simulink model "DroopControl"  (R2025b)
settings: Solver=VariableStepAuto  StartTime=0.0  StopTime=0.3  MaxStep=1/20e3/100  RelTol=1e-3
InitFcn:
  | fs = 20000;
  | Ts = 1/fs;
  | I2B = 10;
  | UB = 20;
  | freq0 = 50;
  | freqc = 0.29999999999999999;
  | w0 = 2*pi*freq0;
  | wc = 2*pi*freqc;
  | I2_Kp = 3.023;
  | I2_Kr = 16.36;
  | Uc_Kp = 0.010579843316015665;
  | Uc_Kr = 0.56544574743993026;
  | I1_Kpi = 1.73;
  | UDC = 48;
  | Ic_Kd = 0;
  | Ts2 = 1/500;
  | 
  | %% 20V / 12A droop-grid configuration
  | % wc_grid is separate from the existing QPR parameter wc.
  | Grid_Condition = 'STRONG'; % STRONG / WEAK_INDUCTIVE / WEAK_RESISTIVE
  | fn = 50;
  | wn = 2*pi*fn;
  | E0 = 20; % phase-voltage peak, V
  | I_base = 12; % current peak, A
  | S_inv = 1.5*E0*I_base;
  | Z_base = E0/I_base;
  | switch Grid_Condition
  |     case 'STRONG'
  |         SCR = 10;
  |         XR_ratio = 5;
  |         Sn = 10*S_inv;
  |         delta_f_max = 0.2;
  |         delta_E_max = 0.02*E0;
  |         grid_wc = 25; % power-filter cutoff, rad/s
  |     case 'WEAK_INDUCTIVE'
  |         SCR = 1.5;
  |         XR_ratio = 3;
  |         Sn = 1.5*S_inv;
  |         delta_f_max = 1.5;
  |         delta_E_max = 0.10*E0;
  |         grid_wc = 120;
  |     case 'WEAK_RESISTIVE'
  |         SCR = 1.5;
  |         XR_ratio = 1;
  |         Sn = 1.5*S_inv;
  |         delta_f_max = 1.5;
  |         delta_E_max = 0.10*E0;
  |         grid_wc = 120;
  |     otherwise
  |         error('DroopGrid:InvalidCondition','Unknown Grid_Condition: %s',Grid_Condition);
  | end
  | Z_grid = Z_base/SCR;
  | Rg_val = Z_grid/sqrt(1+XR_ratio^2);
  | Lg_val = Rg_val*XR_ratio/wn;
  | grid_mp = 2*pi*delta_f_max/Sn;
  | grid_nq = delta_E_max/Sn;
  | grid_p0 = 0;
  | grid_q0 = 0;
  | Ts_ctrl = 1e-4; % actual droop-grid update period, 10 kHz
  | 
  | ... (+21 lines)
model workspace (MAT data in the model file):
  CurrentTestFinalPeak = 0.3
  CurrentTestInitialPeak = 0.1
  CurrentTestSignedStepTime = 0.03
libraries: nesl_utility x31, fl_lib x28, ee_lib x27, simulink x1, eePowerMeasurement x1
(part 2 of 2)

== system DroopControl/I2处理+标幺化/Clark ==
  abc : Inport
  B : Inport  Port=2
  MATLAB Function1 : MATLAB Function  TreatAsAtomicUnit=on
  α : Outport
  β : Outport  Port=2
  wires:
  MATLAB Function1/1(alpha) -> α/1
  abc/1 -> MATLAB Function1/1(abc)
  MATLAB Function1/2(beta) -> β/1
  B/1 -> MATLAB Function1/2(B)

== system DroopControl/数字滤波器+标幺化/Clark1 ==
  abc : Inport
  B : Inport  Port=2
  MATLAB Function1 : MATLAB Function  TreatAsAtomicUnit=on
  α : Outport
  β : Outport  Port=2
  Out3 : Outport  Port=3
  wires:
  MATLAB Function1/1(alpha) -> α/1
  abc/1 -> MATLAB Function1/1(abc)
  MATLAB Function1/2(beta) -> β/1
  B/1 -> MATLAB Function1/2(B)

== system DroopControl/电容线电压处理+标幺化/Clark ==
  abc : Inport
  B : Inport  Port=2
  MATLAB Function1 : MATLAB Function  TreatAsAtomicUnit=on
  α : Outport
  β : Outport  Port=2
  Out3 : Outport  Port=3
  wires:
  B/1 -> MATLAB Function1/2(B)
  MATLAB Function1/2(beta) -> β/1
  abc/1 -> MATLAB Function1/1(abc)
  MATLAB Function1/1(alpha) -> α/1

== system DroopControl/网侧线电压处理+标幺化/Clark ==
  abc : Inport
  B : Inport  Port=2
  MATLAB Function1 : MATLAB Function  TreatAsAtomicUnit=on
  α : Outport
  β : Outport  Port=2
  Out3 : Outport  Port=3
  wires:
  MATLAB Function1/1(alpha) -> α/1
  abc/1 -> MATLAB Function1/1(abc)
  MATLAB Function1/2(beta) -> β/1
  B/1 -> MATLAB Function1/2(B)

== matlab function DroopControl/I2处理+标幺化/Clark/MATLAB Function1 ==
  settings: updateMethod=DISCRETE
  data: abc input; alpha output; beta output; B input
function [alpha, beta] = abc2alphabeta_mux(abc, B)
%#codegen
% ABC2ALPHABETA_MUX  输入 mux 后的 3 通道信号，输出 alpha-beta
%   abc : [3 x N] 矩阵，第 1/2/3 行分别为 a/b/c
%   alpha, beta : [1 x N] 行向量（可直接接 Scope / Mux 输出）
%
%   Simulink 用法：
%     Mux (3 inputs) --> MATLAB Function --> 输出 alpha, beta

    % 按行取出三相，兼容 [3x1] 和 [3xN]
    a = abc(1, :);
    b = abc(2, :);
    c = abc(3, :);

    K = 2/3;   % 等幅值 Clarke 系数；改 sqrt(2/3) 为等功率

    alpha = K * ( a - 0.5*b - 0.5*c ) / B;
    beta  = K * ( (sqrt(3)/2) * (b - c) ) / B;
end

== matlab function DroopControl/Triggered Subsystem1/MATLAB Function1 ==
  settings: updateMethod=DISCRETE
  data: e input; u_r_prev1 input; u_r_prev2 input; e_prev1 input; e_prev2 input; Kp input; Kr input; wc input; w0 input; u_out output; u_r_state output; Ts input
function [u_out, u_r_state] = QPR_Controller(e, u_r_prev1, u_r_prev2, e_prev1, e_prev2, Kp, Kr, wc, w0, Ts)
% QPR电压外环控制器（离散化实现，Tustin变换）
% 输入：
%   e         : 当前时刻电压误差 (v_ref - v_cap)
%   u_r_prev1 : 谐振项上一时刻输出 u_r(k-1)
%   u_r_prev2 : 谐振项上上时刻输出 u_r(k-2)
%   e_prev1   : 上一时刻误差 e(k-1)
%   e_prev2   : 上上时刻误差 e(k-2)
%   Kp, Kr    : 比例系数、谐振系数
%   wc        : 截止频率 (rad/s)
%   w0        : 谐振频率 (rad/s)，如 2*pi*50
%   Ts        : 采样周期 (s)
%
% 输出：
%   u_out     : QPR控制器输出
%   u_r_state : 谐振项当前输出（用于下一时刻状态更新）

% 计算离散化系数
xi = 2 * wc;
den = 4 + 2*xi*Ts + w0^2*Ts^2;

a1 = 2 * (w0^2*Ts^2 - 4) / den;
a2 = (4 - 2*xi*Ts + w0^2*Ts^2) / den;
b0 = 4 * Kr * xi * Ts / den;
b1 = 0;
b2 = -b0;

% 谐振项差分方程迭代
u_r = b0*e + b1*e_prev1 + b2*e_prev2 - a1*u_r_prev1 - a2*u_r_prev2;

% 比例项 + 谐振项
u_out = Kp * e + u_r;

% 输出当前谐振项状态（供下一周期使用）
u_r_state = u_r;
end

== matlab function DroopControl/I1处理+标幺化/Clark/MATLAB Function1 ==
  settings: updateMethod=DISCRETE
  data: abc input; alpha output; beta output; B input
function [alpha, beta] = abc2alphabeta_mux(abc, B)
%#codegen
% ABC2ALPHABETA_MUX  输入 mux 后的 3 通道信号，输出 alpha-beta
%   abc : [3 x N] 矩阵，第 1/2/3 行分别为 a/b/c
%   alpha, beta : [1 x N] 行向量（可直接接 Scope / Mux 输出）
%
%   Simulink 用法：
%     Mux (3 inputs) --> MATLAB Function --> 输出 alpha, beta

    % 按行取出三相，兼容 [3x1] 和 [3xN]
    a = abc(1, :);
    b = abc(2, :);
    c = abc(3, :);

    K = 2/3;   % 等幅值 Clarke 系数；改 sqrt(2/3) 为等功率

    alpha = K * ( a - 0.5*b - 0.5*c ) / B;
    beta  = K * ( (sqrt(3)/2) * (b - c) ) / B;
end

== matlab function DroopControl/I1处理+标幺化/MATLAB Function1 ==
  settings: updateMethod=DISCRETE
  data: y output; real input
function y = fcn(real)
   y = real;
end

== matlab function DroopControl/DroopGridEngine/MATLAB Function1 ==
  settings: updateMethod=DISCRETE  sampleTime=Ts_ctrl
  data: Vabc input; Iabc input; E0 input; wn input; mp input; nq input; wc input; P0 input; Q0 input; v_cmd_abc output; Ts input
function v_cmd_abc = Simscape_Droop_Grid(Vabc, Iabc, E0, wn, mp, nq, wc, P0, Q0, Ts)
%#codegen
% 输入:
%   Vabc      : 采样相电压 [va; vb; vc] (V)
%   Iabc      : 采样输出电流 [ia; ib; ic] (A)
%   E0, wn    : 额定相电压幅值 (V) 与工频角频率 (rad/s)
%   mp, nq    : 下垂系数
%   wc        : 功率低通滤波截止角频率 (rad/s)
%   P0, Q0    : 基准工作功率
%   Ts        : 控制步长 (s)
% 输出:
%   v_cmd_abc : 输送给受控源的参考相电压 [va*; vb*; vc*]

persistent P_filt Q_filt theta
if isempty(P_filt)
    P_filt = 0;
    Q_filt = 0;
    theta = 0;
end

%% 1. 瞬时功率计算 (等幅值 Clarke 变换)
va = Vabc(1); vb = Vabc(2); vc = Vabc(3);
ia = Iabc(1); ib = Iabc(2); ic = Iabc(3);

% Clarke 变换 (2/3 系数)
v_alpha = (2/3) * (va - 0.5 * vb - 0.5 * vc);
v_beta  = (2/3) * (sqrt(3)/2 * vb - sqrt(3)/2 * vc);

i_alpha = (2/3) * (ia - 0.5 * ib - 0.5 * ic);
i_beta  = (2/3) * (sqrt(3)/2 * ib - sqrt(3)/2 * ic);

% 瞬时有功与无功
p_inst = 1.5 * (v_alpha * i_alpha + v_beta * i_beta);
q_inst = 1.5 * (v_beta  * i_alpha - v_alpha * i_beta);

%% 2. 功率滤波 (消除开关纹波并模拟系统惯性)
alpha = (wc * Ts) / (1 + wc * Ts);
P_filt = (1 - alpha) * P_filt + alpha * p_inst;
Q_filt = (1 - alpha) * Q_filt + alpha * q_inst;

%% 3. 下垂特性
w_grid = wn - mp * (P_filt - P0);
E_grid = E0 - nq * (Q_filt - Q0);

% 幅值软限幅防击穿
if E_grid < 0.7 * E0
    E_grid = 0.7 * E0;
elseif E_grid > 1.3 * E0
    E_grid = 1.3 * E0;
end

%% 4. 相角积分
theta = theta + w_grid * Ts;
if theta >= 2 * pi
    theta = theta - 2 * pi;
elseif theta < 0
    theta = theta + 2 * pi;
end

%% 5. 合成三相调制波
v_cmd_abc = [
    E_grid * cos(theta);
    E_grid * cos(theta - 2*pi/3);
    E_grid * cos(theta + 2*pi/3)
];
end

== matlab function DroopControl/Droop Controll /MATLAB Function1 ==
  settings: updateMethod=DISCRETE
  data: v_cap_alpha input; v_cap_beta input; i_inv_alpha input; i_inv_beta input; v_grid_alpha input; v_grid_beta input; w0 input; E0 input; mp input; nq input; wc input; v_alpha_ref output; v_beta_ref output; Ts input; P_filt output; Q_filt output; w_out output; breaker_cmd output
function [v_alpha_ref, v_beta_ref, P_filt, Q_filt, w_out, breaker_cmd] = Droop_Control_Sync( ...
    v_cap_alpha,  v_cap_beta,  ... % 【输入1】逆变器输出电容侧电压 (αβ 坐标系)
    i_inv_alpha,  i_inv_beta,  ... % 【输入2】逆变器输出侧网侧/负载电流 (αβ 坐标系)
    v_grid_alpha, v_grid_beta, ... % 【输入3】外部主电网侧母线电压 (αβ 坐标系)
    w0, E0, mp, nq, wc, Ts)
%#codegen
% =========================================================================
% 输入说明:
%   v_cap_alpha, v_cap_beta   : [输出电容侧] 逆变器 LC 滤波电容两端电压 (V)
%   i_inv_alpha, i_inv_beta   : [输出电容侧] 流向断路器/负载的输出电流 (A)
%   v_grid_alpha, v_grid_beta : [外部电网侧] 三相断路器外侧电网母线电压 (V)
%   w0, E0                    : 额定角频率 (rad/s) 与额定相电压幅值 (V)
%   mp, nq                    : 有功/无功下垂系数
%   wc                        : 功率低通滤波截止角频率 (rad/s)
%   Ts                        : 控制步长 (s)
% 输出说明:
%   v_alpha_ref, v_beta_ref   : QPR 电压内环参考电压 (αβ 轴)
%   P_filt, Q_filt            : 滤波后的有功/无功功率
%   f_out                     : 逆变器当前输出频率 (Hz)
%   breaker_cmd               : 三相断路器合闸指令 (3x1 向量: [cmd_a; cmd_b; cmd_c])
%                               0 = 断开 (未同步/离网), 1 = 合闸导通 (同步完成)
% =========================================================================

%% 内部状态保持
persistent P_prev Q_prev theta_prev
persistent sync_integ sync_ok_counter is_breaker_closed

if isempty(P_prev)
    P_prev = 0;
    Q_prev = 0;
    theta_prev = 0;
    sync_integ = 0;
    sync_ok_counter = 0;
    is_breaker_closed = false;
end

%% 1. 瞬时功率计算 (基于输出电容侧电压与输出电流)
p_inst = 1.5 * (v_cap_alpha * i_inv_alpha + v_cap_beta * i_inv_beta);
q_inst = 1.5 * (v_cap_beta * i_inv_alpha - v_cap_alpha * i_inv_beta);

%% 2. 功率一阶低通滤波
alpha = (wc * Ts) / (1 + wc * Ts);
P_filt = (1 - alpha) * P_prev + alpha * p_inst;
Q_filt = (1 - alpha) * Q_prev + alpha * q_inst;
P_prev = P_filt;
Q_prev = Q_filt;

% 3. Independent inverter: presynchronization and closure disabled.
w_sync = 0;
E_sync = 0;

%% 4. 下垂方程叠加与参考频率/幅值生成
% 频率计算 (并网前叠加上 w_sync 进行调相；并网后 w_sync 归零，由 -mp*P 维持功角自同步)
w_out = (w0 - mp * P_filt) + w_sync;

% 幅值计算 (并网前叠加上 E_sync 消除压差；并网后回归标准下垂)
E_out = (E0 - nq * Q_filt) + E_sync;

% 基础安全限幅
if E_out < 0.8 * E0
    E_out = 0.8 * E0;
elseif E_out > 1.2 * E0
    E_out = 1.2 * E0;
end

%% 5. 相角自累加积分
theta = theta_prev + w_out * Ts;
if theta >= 2 * pi
    theta = theta - 2 * pi;
elseif theta < 0
    theta = theta + 2 * pi;
end
theta_prev = theta;

%% 6. 合成 αβ 轴参考电压 (送入 QPR 电压内环)
v_alpha_ref = E_out * cos(theta);
v_beta_ref  = E_out * sin(theta);

%% 7. 组装三相断路器动作信号
if is_breaker_closed
    % 准同期条件满足，输出合闸指令 (给 1 触发导通/合闸)
    breaker_cmd = [0; 0; 0];
else
    % 预同步中或离网状态，保持断开
    breaker_cmd = [1; 1; 1];
end

end

== matlab function DroopControl/电容线电压处理+标幺化/Clark/MATLAB Function1 ==
  settings: updateMethod=DISCRETE
  data: abc input; alpha output; beta output; B input
function [alpha, beta] = abc2alphabeta_mux(abc, B)
%#codegen
% ABC2ALPHABETA_MUX  输入 mux 后的 3 通道信号，输出 alpha-beta
%   abc : [3 x N] 矩阵，第 1/2/3 行分别为 a/b/c
%   alpha, beta : [1 x N] 行向量（可直接接 Scope / Mux 输出）
%
%   Simulink 用法：
%     Mux (3 inputs) --> MATLAB Function --> 输出 alpha, beta

    % 按行取出三相，兼容 [3x1] 和 [3xN]
    a = abc(1, :);
    b = abc(2, :);
    c = abc(3, :);

    K = 2/3;   % 等幅值 Clarke 系数；改 sqrt(2/3) 为等功率

    alpha = K * ( a - 0.5*b - 0.5*c ) / B;
    beta  = K * ( (sqrt(3)/2) * (b - c) ) / B;
end

== matlab function DroopControl/电容线电压处理+标幺化/MATLAB Function1 ==
  settings: updateMethod=DISCRETE
  data: Uabc output; U_line input
function Uabc = line2phase(U_line)
%#codegen
% 输入 U_line: [Uab; Ubc; Uac]  3x1
% 输出 Uabc : [Ua;  Ub;  Uc ]  3x1

Uab = U_line(1);
Ubc = U_line(2);
Uac = U_line(3);

Ua = ( Uab + Uac) / 3;
Ub = ( Ubc - Uab) / 3;
Uc = -(Ubc + Uac) / 3;

Uabc = [Ua; Ub; Uc];
end

== matlab function DroopControl/Triggered Subsystem2/MATLAB Function1 ==
  settings: updateMethod=DISCRETE
  data: i1_alpha_ref input; i1_beta_ref input; i1_alpha input; i1_beta input; uc_alpha input; uc_beta input; Kpi input; u_alpha_ref output; u_beta_ref output
function [u_alpha_ref, u_beta_ref] = current_loop( ...
    i1_alpha_ref, i1_beta_ref, ...
    i1_alpha, i1_beta, ...
    uc_alpha, uc_beta, Kpi)
%#codegen
% i1 比例电流环，带 uc 电压前馈，不加 ic 阻尼
%
% 电流单位：A
% 电压单位：V
% Kpi 单位：V/A（欧姆）
% 输出：送往调制器的 alpha、beta 电压指令

% 电流误差
e_alpha = i1_alpha_ref - i1_alpha;
e_beta  = i1_beta_ref  - i1_beta;

% 比例控制 + 电容电压前馈
u_alpha_ref = Kpi * e_alpha + uc_alpha;
u_beta_ref  = Kpi * e_beta  + uc_beta;

end

== matlab function DroopControl/α,β转SVPWM调制波1/MATLAB Function1 ==
  settings: updateMethod=DISCRETE
  data: valpha_pu input; A_SVM output; B_SVM output; vbeta_pu input; C_SVM output; Vbase input; Udc input
function [A_SVM, B_SVM, C_SVM] = ...
    svpwm_simple_pu(valpha_pu, vbeta_pu, Vbase, Udc)
%#codegen

% 母线电压尚未建立时，输出零线电压指令
if Udc <= 1e-6
    A_SVM = 0;
    B_SVM = 0;
    C_SVM = 0;
    return;
end

% 将控制器输出恢复为实际电压
Va = valpha_pu * Vbase;
Vb = vbeta_pu  * Vbase;

% 反 Clarke 变换
v = [Va, (-Va + sqrt(3)*Vb)/2, ...
         (-Va - sqrt(3)*Vb)/2];

% 超出母线可实现范围时，等比例缩小电压矢量
span = max(v) - min(v);
if span > Udc
    v = v * (Udc / span);
end

% 零序注入，转换为 0～1 上管占空比
v0 = (max(v) + min(v)) / 2;
d = 0.5 + (v - v0) / Udc;
d = min(max(d, 0), 1);

A_SVM = 2*d(1)-1;
B_SVM = 2*d(2)-1;
C_SVM = 2*d(3)-1;
end
% Average converter ModWave uses signed modulation m=2*d-1.

== matlab function DroopControl/数字滤波器+标幺化/Clark1/MATLAB Function1 ==
  settings: updateMethod=DISCRETE
  data: abc input; alpha output; beta output; B input
function [alpha, beta] = abc2alphabeta_mux(abc, B)
%#codegen
% ABC2ALPHABETA_MUX  输入 mux 后的 3 通道信号，输出 alpha-beta
%   abc : [3 x N] 矩阵，第 1/2/3 行分别为 a/b/c
%   alpha, beta : [1 x N] 行向量（可直接接 Scope / Mux 输出）
%
%   Simulink 用法：
%     Mux (3 inputs) --> MATLAB Function --> 输出 alpha, beta

    % 按行取出三相，兼容 [3x1] 和 [3xN]
    a = abc(1, :);
    b = abc(2, :);
    c = abc(3, :);

    K = 2/3;   % 等幅值 Clarke 系数；改 sqrt(2/3) 为等功率

    alpha = K * ( a - 0.5*b - 0.5*c ) / B;
    beta  = K * ( (sqrt(3)/2) * (b - c) ) / B;
end

== matlab function DroopControl/I2处理+标幺化/MATLAB Function1 ==
  settings: updateMethod=DISCRETE
  data: y output; real input
function y = fcn(real)
   y = real;
end

== matlab function DroopControl/网侧线电压处理+标幺化/MATLAB Function1 ==
  settings: updateMethod=DISCRETE
  data: Uabc output; U_line input
function Uabc = line2phase(U_line)
%#codegen
% 输入 U_line: [Uab; Ubc; Uac]  3x1
% 输出 Uabc : [Ua;  Ub;  Uc ]  3x1

Uab = U_line(1);
Ubc = U_line(2);
Uac = U_line(3);

Ua = ( Uab + Uac) / 3;
Ub = ( Ubc - Uab) / 3;
Uc = -(Ubc + Uac) / 3;

Uabc = [Ua; Ub; Uc];
end

== matlab function DroopControl/数字滤波器+标幺化/MATLAB Function1 ==
  settings: updateMethod=DISCRETE
  data: y output; real input
function y = fcn(real)
   y = real;
end

== matlab function DroopControl/θ转α,β/MATLAB Function1 ==
  settings: updateMethod=DISCRETE
  data: theta input; alpha output; beta output
function [alpha, beta] = theta2alphabeta(theta)
%#codegen
% 输入 theta: 电角度 (rad)
% 输出 alpha, beta: αβ 分量

alpha = cos(theta);
beta  = sin(theta);

end

== matlab function DroopControl/网侧线电压处理+标幺化/Clark/MATLAB Function1 ==
  settings: updateMethod=DISCRETE
  data: abc input; alpha output; beta output; B input
function [alpha, beta] = abc2alphabeta_mux(abc, B)
%#codegen
% ABC2ALPHABETA_MUX  输入 mux 后的 3 通道信号，输出 alpha-beta
%   abc : [3 x N] 矩阵，第 1/2/3 行分别为 a/b/c
%   alpha, beta : [1 x N] 行向量（可直接接 Scope / Mux 输出）
%
%   Simulink 用法：
%     Mux (3 inputs) --> MATLAB Function --> 输出 alpha, beta

    % 按行取出三相，兼容 [3x1] 和 [3xN]
    a = abc(1, :);
    b = abc(2, :);
    c = abc(3, :);

    K = 2/3;   % 等幅值 Clarke 系数；改 sqrt(2/3) 为等功率

    alpha = K * ( a - 0.5*b - 0.5*c ) / B;
    beta  = K * ( (sqrt(3)/2) * (b - c) ) / B;
end

== matlab function DroopControl/SOGI-FLL Subsystem3/MATLAB Function1 ==
  settings: updateMethod=DISCRETE
  data: u input; theta output; omega output; Ts input; locked output
function [theta, omega, locked] = DSOGI_FLL(u, Ts)
% DSOGI-FLL (输入为Mux后的三相电压向量)
% 输入:
%   u  - 3x1 向量 [Ua; Ub; Uc]
%   Ts - 采样周期 (全局变量, 从工作区传入)
% 输出:
%   theta  - 估计相角 (rad)
%   omega  - 估计角频率 (rad/s)
%   locked - 锁相状态 (0=未锁定, 1=已锁定)

% --- 持久变量 (状态) ---
persistent x1_alpha x2_alpha x1_beta x2_beta omega_est lock_cnt
if isempty(x1_alpha)
    x1_alpha = 0; x2_alpha = 0;
    x1_beta  = 0; x2_beta  = 0;
    omega_est = 2*pi*50;   % 初始频率 50 Hz
    lock_cnt  = 0;
end

% --- 参数 ---
k      = sqrt(2);        % SOGI 增益
Gamma  = 100;            % FLL 增益
omega_n = 2*pi*50;       % 额定角频率

% --- 锁定判据参数 ---
eps_lock   = 5;          % 归一化频率误差阈值
lock_hold  = round(0.02 / Ts);   % 连续满足时间 = 20ms 判定为锁定

% --- 1) Clarke 变换 (等幅值) ---
Ua = u(1);  Ub = u(2);  Uc = u(3);
ualpha = (2/3) * (Ua - 0.5*Ub - 0.5*Uc);
ubeta  = (2/3) * ( (sqrt(3)/2)*Ub - (sqrt(3)/2)*Uc );

% --- 2) 限幅保护 ---
omega_est = max(min(omega_est, 2*pi*65), 2*pi*45);

% --- 3) SOGI 离散化 (后向欧拉) ---
% alpha 轴
err_a  = ualpha - x1_alpha;
x1_alpha = x1_alpha + Ts * (k * err_a - x2_alpha) * omega_est;
x2_alpha = x2_alpha + Ts * (x1_alpha * omega_est);

% beta 轴
err_b  = ubeta - x1_beta;
x1_beta = x1_beta + Ts * (k * err_b - x2_beta) * omega_est;
x2_beta = x2_beta + Ts * (x1_beta * omega_est);

% --- 4) 正序分量 (Lyon变换简化形式) ---
v_alpha_pos = 0.5 * (x1_alpha - x2_beta);
v_beta_pos  = 0.5 * (x1_beta  + x2_alpha);

% --- 5) FLL 频率估计 ---
epsilon_f = v_alpha_pos * (x1_beta - ubeta) - v_beta_pos * (x1_alpha - ualpha);

% 归一化 (使 Gamma 与电压幅值无关)
norm_factor = v_alpha_pos^2 + v_beta_pos^2;
if norm_factor > 1e-6
    epsilon_f = epsilon_f / norm_factor;
end
omega_est = omega_est - Gamma * epsilon_f * Ts;

% --- 6) 相角输出 ---
theta = atan2(v_beta_pos, v_alpha_pos);
omega = omega_est;

% --- 7) 锁相完成状态判定 ---
if abs(epsilon_f) < eps_lock
    lock_cnt = lock_cnt + 1;
    if lock_cnt >= lock_hold
        lock_cnt = lock_hold;   % 饱和,防止溢出
    end
else
    lock_cnt = 0;               % 一旦失锁立即清零
end
locked = double(lock_cnt >= lock_hold);

end

== matlab function DroopControl/Triggered Subsystem4/MATLAB Function1 ==
  settings: updateMethod=DISCRETE
  data: e input; u_r_prev1 input; u_r_prev2 input; e_prev1 input; e_prev2 input; Kp input; Kr input; wc input; w0 input; u_out output; u_r_state output; Ts input
function [u_out, u_r_state] = QPR_Controller(e, u_r_prev1, u_r_prev2, e_prev1, e_prev2, Kp, Kr, wc, w0, Ts)
% QPR电压外环控制器（离散化实现，Tustin变换）
% 输入：
%   e         : 当前时刻电压误差 (v_ref - v_cap)
%   u_r_prev1 : 谐振项上一时刻输出 u_r(k-1)
%   u_r_prev2 : 谐振项上上时刻输出 u_r(k-2)
%   e_prev1   : 上一时刻误差 e(k-1)
%   e_prev2   : 上上时刻误差 e(k-2)
%   Kp, Kr    : 比例系数、谐振系数
%   wc        : 截止频率 (rad/s)
%   w0        : 谐振频率 (rad/s)，如 2*pi*50
%   Ts        : 采样周期 (s)
%
% 输出：
%   u_out     : QPR控制器输出
%   u_r_state : 谐振项当前输出（用于下一时刻状态更新）

% 计算离散化系数
xi = 2 * wc;
den = 4 + 2*xi*Ts + w0^2*Ts^2;

a1 = 2 * (w0^2*Ts^2 - 4) / den;
a2 = (4 - 2*xi*Ts + w0^2*Ts^2) / den;
b0 = 4 * Kr * xi * Ts / den;
b1 = 0;
b2 = -b0;

% 谐振项差分方程迭代
u_r = b0*e + b1*e_prev1 + b2*e_prev2 - a1*u_r_prev1 - a2*u_r_prev2;

% 比例项 + 谐振项
u_out = Kp * e + u_r;

% 输出当前谐振项状态（供下一周期使用）
u_r_state = u_r;
end
